simulink model "Motor_Mixing_Bounded"  (R2026b)
settings: Solver=FixedStepDiscrete  FixedStep=0.01
model workspace (MAT data in the model file):
  D = 0.209999993443
  F_max_test = 2
  K_mix = [0.25  -3.36717510223  -3.36717510223  0; 0.25  -3.36717510223  3.36717510223  0; 0.25  3.36717510223  -3.36717510223  0; 0.25  3.36717510223  3.36717510223  0]
  L = 0.104999996722
  d = 0.0742462128401

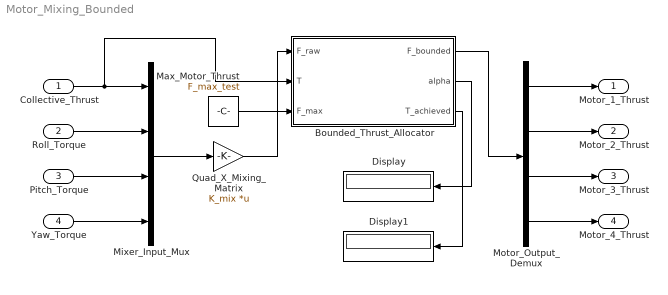
== system Motor_Mixing_Bounded ==
  Collective_Thrust : Inport  OutDataTypeStr=single
  Roll_Torque : Inport  Port=2  OutDataTypeStr=single
  Pitch_Torque : Inport  Port=3  OutDataTypeStr=single
  Yaw_Torque : Inport  Port=4  OutDataTypeStr=single
  Bounded_Thrust_Allocator : MATLAB Function  TreatAsAtomicUnit=on
  Display : Display
  Display1 : Display
  Max_Motor_Thrust : Constant  Value=F_max_test  OutDataTypeStr=single
  Mixer_Input_Mux : Mux
  Motor_Output_Demux : Demux
  Quad_X_Mixing_Matrix : Gain  Gain=K_mix  Multiplication=Matrix(K*u)
  Motor_1_Thrust : Outport
  Motor_2_Thrust : Outport  Port=2
  Motor_3_Thrust : Outport  Port=3
  Motor_4_Thrust : Outport  Port=4
  wires:
  Collective_Thrust/1 -> Bounded_Thrust_Allocator/2(T), Mixer_Input_Mux/1
  Roll_Torque/1 -> Mixer_Input_Mux/2
  Pitch_Torque/1 -> Mixer_Input_Mux/3
  Yaw_Torque/1 -> Mixer_Input_Mux/4
  Mixer_Input_Mux/1 -> Quad_X_Mixing_Matrix/1
  Motor_Output_Demux/1 -> Motor_1_Thrust/1
  Motor_Output_Demux/2 -> Motor_2_Thrust/1
  Motor_Output_Demux/3 -> Motor_3_Thrust/1
  Motor_Output_Demux/4 -> Motor_4_Thrust/1
  Quad_X_Mixing_Matrix/1 -> Bounded_Thrust_Allocator/1(F_raw)
  Bounded_Thrust_Allocator/1(F_bounded) -> Motor_Output_Demux/1
  Max_Motor_Thrust/1 -> Bounded_Thrust_Allocator/3(F_max)
  Bounded_Thrust_Allocator/2(alpha) -> Display/1
  Bounded_Thrust_Allocator/3(T_achieved) -> Display1/1

== matlab function Motor_Mixing_Bounded/Bounded_Thrust_Allocator ==
  data: F_raw input; F_bounded output; T input; F_max input; alpha output; T_achieved output
function [F_bounded, alpha, T_achieved] = ...
    limit_thrust_bounds(F_raw, T, F_max)
%#codegen
% Quad-X Bounded Thrust Allocation
%
% Inputs:
% F_raw : Raw motor thrust vector [4x1] (N)
% T     : Requested collective thrust (N)
% F_max : Maximum thrust per motor (N)
%
% Outputs:
% F_bounded  : Bounded motor thrust [4x1] (N)
% alpha      : Torque correction scale factor
% T_achieved : Achieved collective thrust (N)
%
% Assumptions:
% - Symmetric Quad-X
% - Yaw mixing disabled
% - Minimum thrust = 0 N
% - Identical maximum thrust for all motors

F_bounded = zeros(4, 1, 'single');
alpha = single(0);
T_achieved = single(0);

% Validate input
if ~isfinite(T) || ~isfinite(F_max) || ...
        F_max <= single(0) || any(~isfinite(F_raw))
    return;
end

% Limit collective thrust to feasible range
T_cmd = min(max(T, single(0)), single(4) * F_max);

% Equal thrust distribution
base = T_cmd / single(4);

% Differential thrust from Roll/Pitch
delta = F_raw(:) - T / single(4);

% Remove numerical sum error
delta = delta - sum(delta) / single(4);

% Default correction scale
alpha = single(1);

% Find feasible correction scale
for i = 1:4

    if delta(i) > single(0)

        % Upper thrust constraint
        alpha_i = (F_max - base) / delta(i);
        alpha = min(alpha, alpha_i);

    elseif delta(i) < single(0)

        % Lower thrust constraint
        alpha_i = base / (-delta(i));
        alpha = min(alpha, alpha_i);

    end

end

% Limit alpha to [0, 1]
alpha = min(max(alpha, single(0)), single(1));

% Apply bounded motor thrust
for i = 1:4

    F_bounded(i) = base + alpha * delta(i);

    % Numerical safety clamp
    F_bounded(i) = min( ...
        max(F_bounded(i), single(0)), F_max);

end

% Actual achieved collective thrust
T_achieved = sum(F_bounded);

end
